simulink model "sensorExpoler"  (R2026a)
settings: Solver=FixedStepDiscrete  StopTime=30  FixedStep=0.001
undefined symbols (not defined in the file or in its folder): Blocking, Non
libraries: amg_usbconverter_n_connect_lib x2
settings Model: Creator=pboon  LastModifiedBy=rosva

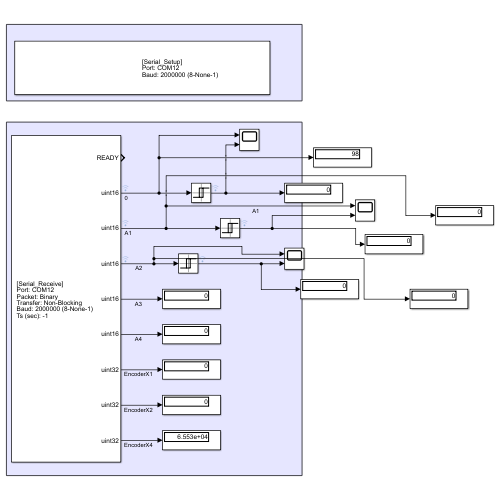
[thumbnail: Simulink's stored preview of the top-level diagram]
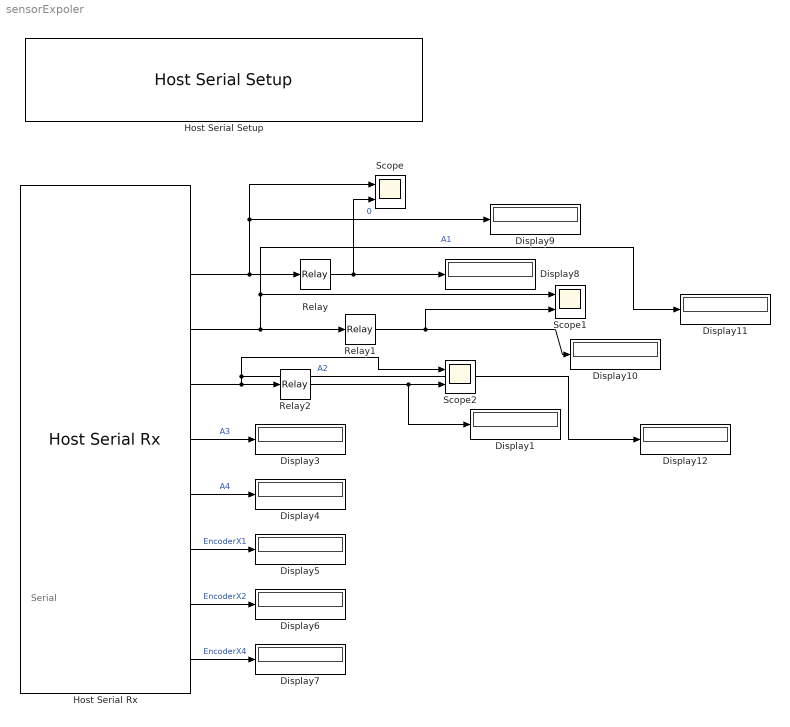
== system sensorExpoler ==
  note: Serial
  Display{1,3..12} (11 alike) : Display
  Host Serial Rx : amg_usbconverter_n_connect_lib/Host Serial Rx  conf=rx  port=COM12  baudrate=2000000  databits=8  parity=None  stopbit=1  flowcontrol=None  transfer=Non-Blocking  timeout=5  packetmode=Binary  enableinitialvalues=off  initialvalues=[]  binheader='25'  binterminator='4E 4E'  porttype_double=0  porttype_single=0  porttype_int8=0  porttype_uint8=0  porttype_int16=0  porttype_uint16=5  porttype_int32=0  porttype_uint32=3  asciiformat='%d,%f'  rx_asciiterminator="CRLF (0x0D 0x0A - \"\\r\\n\")"  tx_asciiterminator="CRLF (0x0D 0x0A - \"\\r\\n\")"  sampletime=0.001  enablecustomportlabel=off  cinputportlabel=0  coutputportlabel=A  portpinstr=0  blockid=HostSerialRx  inputporttype=[]  inputportwidth=[]  inputportlabel={}  outputporttype=[3 5 5 5 5 5 7 7 7]  outputportwidth=[1 1 1 1 1 1 1 1 1]  outputportlabel={'READY','uint16','uint16','uint16','uint16','uint16','uint32','uint32','uint32'}  compat=0  optionstring=[]  autoport='COM12'
  Host Serial Setup : amg_usbconverter_n_connect_lib/Host Serial Setup  conf=setup  port=COM12  baudrate=2000000  databits=8  parity=None  stopbit=1  flowcontrol=None  transfer=Blocking  timeout=2  packetmode=Binary  initialvalues=[]  binheader='7E 7E'  binterminator='03 03'  porttype_double=0  porttype_single=1  porttype_int8=0  porttype_uint8=0  porttype_int16=0  porttype_uint16=0  porttype_int32=0  porttype_uint32=2  asciiformat='%d %u %x'  rx_asciiterminator="CRLF (0x0D 0x0A - \"\\r\\n\")"  tx_asciiterminator="CRLF (0x0D 0x0A - \"\\r\\n\")"  sampletime=-1  enablecustomportlabel=off  cinputportlabel=0  coutputportlabel=A  portpinstr=0  blockid=HostSerialSetup  inputporttype=[]  inputportwidth=[]  inputportlabel={}  outputporttype=[]  outputportwidth=[]  outputportlabel={}  compat=0  optionstring=[]  autoport='COM12'
  Relay : Relay  OnSwitchValue=2500  OffSwitchValue=1000
  Relay1 : Relay  OnSwitchValue=2500  OffSwitchValue=1000
  Relay2 : Relay  OnSwitchValue=2500  OffSwitchValue=1000
  Scope : Scope  NumInputPorts=2
      settings: ActiveDisplayYMinimum=-205.34499632319498  ActiveDisplayYMaximum=304.85079094439152
  Scope1 : Scope  NumInputPorts=2
      settings: ActiveDisplayYMinimum=-205.34499632319498  ActiveDisplayYMaximum=304.85079094439152
  Scope2 : Scope  NumInputPorts=2
      settings: ActiveDisplayYMinimum=-205.34499632319498  ActiveDisplayYMaximum=304.85079094439152  DataLoggingVariableName=ScopeData2
  wires:
  Host Serial Rx/3 -> Display11/1, Scope1/1, Relay1/1  "A1"
  Host Serial Rx/4 -> Scope2/1, Display12/1, Relay2/1  "A2"
  Host Serial Rx/5 -> Display3/1  "A3"
  Host Serial Rx/6 -> Display4/1  "A4"
  Host Serial Rx/7 -> Display5/1  "EncoderX1"
  Host Serial Rx/8 -> Display6/1  "EncoderX2"
  Host Serial Rx/9 -> Display7/1  "EncoderX4"
  Host Serial Rx/2 -> Scope/1, Display9/1, Relay/1  "0"
  Relay/1 -> Display8/1, Scope/2
  Relay1/1 -> Display10/1, Scope1/2
  Relay2/1 -> Scope2/2, Display1/1
